simulink library "RS50_20S6P"  (R2025b)
settings: Solver=VariableStepAuto  StartTime=0.0  StopTime=10.0  RelTol=1e-3
undefined symbols (not defined in the file or in its folder): battery_builder_rtmsupport, gcbh
libraries: RS50_20S6P_lib x6
settings Model: Creator=oscar  LastModifiedBy=oscar

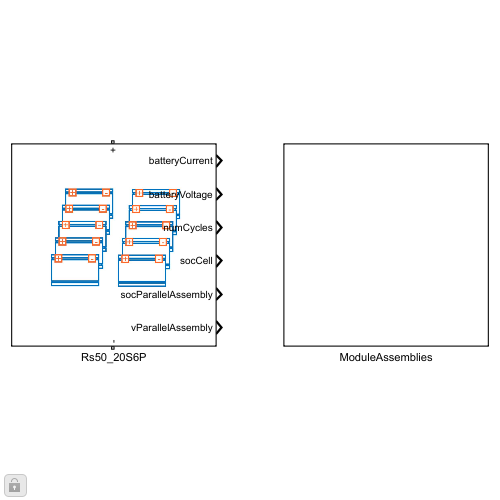
[thumbnail: Simulink's stored preview of the top-level diagram]
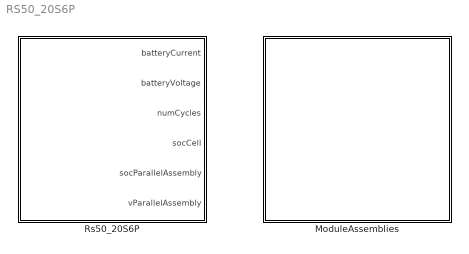
== system RS50_20S6P ==
  ModuleAssemblies : Subsystem
  Rs50_20S6P : Subsystem  LoadFcn=battery_builder_rtmsupport('loadfcn',gcbh);
      settings: CopyFcn=battery_builder_rtmsupport('copyfcn',gcbh);  PreCopyFcn=battery_builder_rtmsupport('precopyfcn',gcbh);  PreDeleteFcn=battery_builder_rtmsupport('predeletefcn',gcbh);  PortSchema="{\"entries\":[{\"content\":{\"sides\":[{\"content\":{\"connectorIds\":[\"LConn1\"]},\"type\":\"ConnectorPlacement.EquallySpacedRectSide\",\"uuid\":\"68108b1f-35ee-4bf1-8cf0-16152839d0de\"},{\"content\":{\"connectorIds\":[\"RConn1\"],\"side\":\"RIGHT\"},\"type\":\"ConnectorPlacement.EquallySpacedRectSide\",\"uuid\":\"9025f6ce-e211-4c4c-af6a-c12758361a55\"},{\"content\":{\"side\":\"TOP\"},\"type\":\"ConnectorPlacement.EquallySpacedRectSide\",\"uuid\":\"21b2816d-4a17-450d-8c21-7c5f468b8140\"},{\"content\":{\"connectorIds\":[\"Out1\",\"Out2\",\"Out3\",\"Out4\",\"Out5\",\"Out6\"],\"side\":\"BOTTOM\"},\"type\":\"ConnectorPlacement.EquallySpacedRectSide\",\"uuid\":\"2d886023-0113-46b2-8405-f6ad4fc498bb\"}]},\"type\":\"ConnectorPlacement.EquallySpacedConnector\",\"uuid\":\"b4619561-6c89-449f-a42b-64cd7bd240c0\"}],\"packageUris\":[\"http://schema.mathworks.com/mf0/Connector/R2020b\"],\"version\":\"1.0\"}"
      mask Display: image('$imagefile')

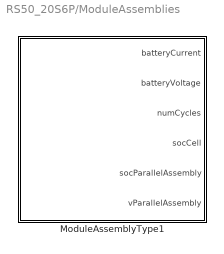
== system RS50_20S6P/ModuleAssemblies ==
  ModuleAssemblyType1 : Subsystem  LoadFcn=battery_builder_rtmsupport('loadfcn',gcbh);
      settings: CopyFcn=battery_builder_rtmsupport('copyfcn',gcbh);  PreCopyFcn=battery_builder_rtmsupport('precopyfcn',gcbh);  PreDeleteFcn=battery_builder_rtmsupport('predeletefcn',gcbh);  PortSchema="{\"entries\":[{\"content\":{\"sides\":[{\"content\":{\"connectorIds\":[\"LConn1\"]},\"type\":\"ConnectorPlacement.EquallySpacedRectSide\",\"uuid\":\"68108b1f-35ee-4bf1-8cf0-16152839d0de\"},{\"content\":{\"connectorIds\":[\"RConn1\"],\"side\":\"RIGHT\"},\"type\":\"ConnectorPlacement.EquallySpacedRectSide\",\"uuid\":\"9025f6ce-e211-4c4c-af6a-c12758361a55\"},{\"content\":{\"side\":\"TOP\"},\"type\":\"ConnectorPlacement.EquallySpacedRectSide\",\"uuid\":\"21b2816d-4a17-450d-8c21-7c5f468b8140\"},{\"content\":{\"connectorIds\":[\"Out1\",\"Out2\",\"Out3\",\"Out4\",\"Out5\",\"Out6\"],\"side\":\"BOTTOM\"},\"type\":\"ConnectorPlacement.EquallySpacedRectSide\",\"uuid\":\"a11e89a2-602c-4dcc-bda4-f5b907a63c99\"}]},\"type\":\"ConnectorPlacement.EquallySpacedConnector\",\"uuid\":\"b4619561-6c89-449f-a42b-64cd7bd240c0\"}],\"packageUris\":[\"http://schema.mathworks.com/mf0/Connector/R2020b\"],\"version\":\"1.0\"}"
      mask Display: image('$imagefile')

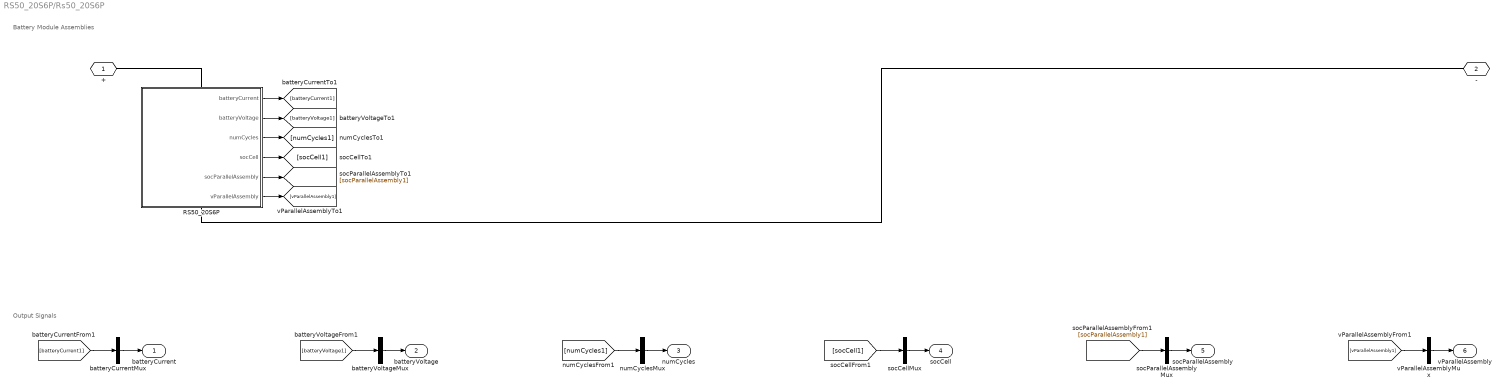
== system RS50_20S6P/Rs50_20S6P ==
  note: Battery Module Assemblies
  note: Output Signals
  RS50_20S6P : Subsystem  LoadFcn=battery_builder_rtmsupport('loadfcn',gcbh);
      settings: CopyFcn=battery_builder_rtmsupport('copyfcn',gcbh);  PreCopyFcn=battery_builder_rtmsupport('precopyfcn',gcbh);  PreDeleteFcn=battery_builder_rtmsupport('predeletefcn',gcbh);  PortSchema="{\"entries\":[{\"content\":{\"sides\":[{\"content\":{\"connectorIds\":[\"LConn1\"]},\"type\":\"ConnectorPlacement.EquallySpacedRectSide\",\"uuid\":\"68108b1f-35ee-4bf1-8cf0-16152839d0de\"},{\"content\":{\"connectorIds\":[\"RConn1\"],\"side\":\"RIGHT\"},\"type\":\"ConnectorPlacement.EquallySpacedRectSide\",\"uuid\":\"9025f6ce-e211-4c4c-af6a-c12758361a55\"},{\"content\":{\"side\":\"TOP\"},\"type\":\"ConnectorPlacement.EquallySpacedRectSide\",\"uuid\":\"21b2816d-4a17-450d-8c21-7c5f468b8140\"},{\"content\":{\"connectorIds\":[\"Out1\",\"Out2\",\"Out3\",\"Out4\",\"Out5\",\"Out6\"],\"side\":\"BOTTOM\"},\"type\":\"ConnectorPlacement.EquallySpacedRectSide\",\"uuid\":\"a11e89a2-602c-4dcc-bda4-f5b907a63c99\"}]},\"type\":\"ConnectorPlacement.EquallySpacedConnector\",\"uuid\":\"b4619561-6c89-449f-a42b-64cd7bd240c0\"}],\"packageUris\":[\"http://schema.mathworks.com/mf0/Connector/R2020b\"],\"version\":\"1.0\"}"
      mask Display: image('$imagefile')
  batteryCurrentMux : Mux  Inputs=1
  batteryVoltageMux : Mux  Inputs=1
  numCyclesMux : Mux  Inputs=1
  socCellMux : Mux  Inputs=1
  socParallelAssemblyMux : Mux  Inputs=1
  vParallelAssemblyMux : Mux  Inputs=1
  + : PMIOPort  Side=Left
  - : PMIOPort  Port=2  Side=Right
  batteryCurrent : Outport
  batteryVoltage : Outport  Port=2
  numCycles : Outport  Port=3
  socCell : Outport  Port=4
  socParallelAssembly : Outport  Port=5
  vParallelAssembly : Outport  Port=6
  wires:
  RS50_20S6P/1(batteryCurrent) -> [batteryCurrent1]
  batteryCurrentMux/1 -> batteryCurrent/1
  [batteryCurrent1] -> batteryCurrentMux/1
  RS50_20S6P/2(batteryVoltage) -> [batteryVoltage1]
  batteryVoltageMux/1 -> batteryVoltage/1
  [batteryVoltage1] -> batteryVoltageMux/1
  RS50_20S6P/3(numCycles) -> [numCycles1]
  numCyclesMux/1 -> numCycles/1
  [numCycles1] -> numCyclesMux/1
  RS50_20S6P/4(socCell) -> [socCell1]
  socCellMux/1 -> socCell/1
  [socCell1] -> socCellMux/1
  RS50_20S6P/5(socParallelAssembly) -> [socParallelAssembly1]
  socParallelAssemblyMux/1 -> socParallelAssembly/1
  [socParallelAssembly1] -> socParallelAssemblyMux/1
  RS50_20S6P/6(vParallelAssembly) -> [vParallelAssembly1]
  vParallelAssemblyMux/1 -> vParallelAssembly/1
  [vParallelAssembly1] -> vParallelAssemblyMux/1
  connections:
  RS50_20S6P/LConn1 -- +/RConn1
  RS50_20S6P/RConn1 -- -/RConn1

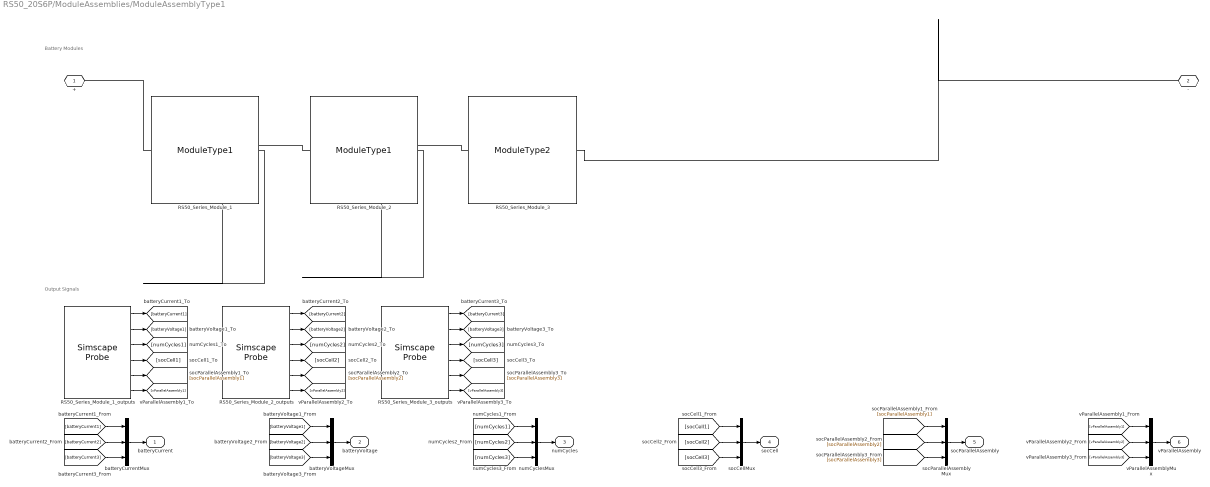
== system RS50_20S6P/ModuleAssemblies/ModuleAssemblyType1 ==
  note: Battery Modules
  note: Output Signals
  RS50_Series_Module_1 : RS50_20S6P_lib/Modules/ModuleType1  BatteryCapacityCell=27 A*hr  ExtrapolationMethodCell=simscape.enum.extrapolation.nearest  SOCBreakpointsCell=[0, .1, .25, .5, .75, .9, 1]  OpenCircuitVoltageCell=[3.5057, 3.566, 3.6337, 3.7127, 3.9259, 4.0777, 4.1928] V  VoltageRangeCell=[0, inf] V  ResistanceSOCBreakpointsCell=[0, .1, .25, .5, .75, .9, 1]  R0Cell=[.0085, .0085, .0087, .0082, .0083, .0085, .0085] Ohm  P=6  S=7  socCell_specify=off  socCell_priority=High  socCell=1  socCell_nominal_specify=off  socCell_nominal_value=1  socCell_nominal_unit=1  batteryVoltage_specify=off  batteryVoltage_priority=None  batteryVoltage=0 V  batteryVoltage_nominal_specify=off  batteryVoltage_nominal_value=1  batteryVoltage_nominal_unit=V  batteryCurrent_specify=off  batteryCurrent_priority=None  batteryCurrent=0 A  batteryCurrent_nominal_specify=off  batteryCurrent_nominal_value=1  batteryCurrent_nominal_unit=A  numCycles_specify=off  numCycles_priority=High  numCycles=0  numCycles_nominal_specify=off  numCycles_nominal_value=1  numCycles_nominal_unit=1  vParallelAssembly_specify=off  vParallelAssembly_priority=None  vParallelAssembly=repmat(0, 7, 1) V  vParallelAssembly_nominal_specify=off  vParallelAssembly_nominal_value=1  vParallelAssembly_nominal_unit=V  socParallelAssembly_specify=off  socParallelAssembly_priority=None  socParallelAssembly=repmat(1, 7, 1)  socParallelAssembly_nominal_specify=off  socParallelAssembly_nominal_value=1  socParallelAssembly_nominal_unit=1
      settings: InternalSimscapePortConfiguration="{\"Bottom\":[{\"id\":\"n\",\"label\":\"-\",\"type\":\"foundation.electrical.electrical\"}],\"Left\":[],\"Right\":[],\"Top\":[{\"id\":\"p\",\"label\":\"+\",\"type\":\"foundation.electrical.electrical\"}]}"
  RS50_Series_Module_1_outputs : SimscapeProbe  BoundBlock=3  Variables="{\"batteryCurrent\":{\"Probing\":\"ON\"},\"batteryVoltage\":{\"Probing\":\"ON\"},\"numCycles\":{\"Probing\":\"ON\"},\"socCell\":{\"Probing\":\"ON\"},\"socParallelAssembly\":{\"Probing\":\"ON\"},\"vParallelAssembly\":{\"Probing\":\"ON\"}}"
  RS50_Series_Module_2 : RS50_20S6P_lib/Modules/ModuleType1  BatteryCapacityCell=27 A*hr  ExtrapolationMethodCell=simscape.enum.extrapolation.nearest  SOCBreakpointsCell=[0, .1, .25, .5, .75, .9, 1]  OpenCircuitVoltageCell=[3.5057, 3.566, 3.6337, 3.7127, 3.9259, 4.0777, 4.1928] V  VoltageRangeCell=[0, inf] V  ResistanceSOCBreakpointsCell=[0, .1, .25, .5, .75, .9, 1]  R0Cell=[.0085, .0085, .0087, .0082, .0083, .0085, .0085] Ohm  P=6  S=7  socCell_specify=off  socCell_priority=High  socCell=1  socCell_nominal_specify=off  socCell_nominal_value=1  socCell_nominal_unit=1  batteryVoltage_specify=off  batteryVoltage_priority=None  batteryVoltage=0 V  batteryVoltage_nominal_specify=off  batteryVoltage_nominal_value=1  batteryVoltage_nominal_unit=V  batteryCurrent_specify=off  batteryCurrent_priority=None  batteryCurrent=0 A  batteryCurrent_nominal_specify=off  batteryCurrent_nominal_value=1  batteryCurrent_nominal_unit=A  numCycles_specify=off  numCycles_priority=High  numCycles=0  numCycles_nominal_specify=off  numCycles_nominal_value=1  numCycles_nominal_unit=1  vParallelAssembly_specify=off  vParallelAssembly_priority=None  vParallelAssembly=repmat(0, 7, 1) V  vParallelAssembly_nominal_specify=off  vParallelAssembly_nominal_value=1  vParallelAssembly_nominal_unit=V  socParallelAssembly_specify=off  socParallelAssembly_priority=None  socParallelAssembly=repmat(1, 7, 1)  socParallelAssembly_nominal_specify=off  socParallelAssembly_nominal_value=1  socParallelAssembly_nominal_unit=1
      settings: InternalSimscapePortConfiguration="{\"Bottom\":[{\"id\":\"n\",\"label\":\"-\",\"type\":\"foundation.electrical.electrical\"}],\"Left\":[],\"Right\":[],\"Top\":[{\"id\":\"p\",\"label\":\"+\",\"type\":\"foundation.electrical.electrical\"}]}"
  RS50_Series_Module_2_outputs : SimscapeProbe  BoundBlock=4  Variables="{\"batteryCurrent\":{\"Probing\":\"ON\"},\"batteryVoltage\":{\"Probing\":\"ON\"},\"numCycles\":{\"Probing\":\"ON\"},\"socCell\":{\"Probing\":\"ON\"},\"socParallelAssembly\":{\"Probing\":\"ON\"},\"vParallelAssembly\":{\"Probing\":\"ON\"}}"
  RS50_Series_Module_3 : RS50_20S6P_lib/Modules/ModuleType2  BatteryCapacityCell=27 A*hr  ExtrapolationMethodCell=simscape.enum.extrapolation.nearest  SOCBreakpointsCell=[0, .1, .25, .5, .75, .9, 1]  OpenCircuitVoltageCell=[3.5057, 3.566, 3.6337, 3.7127, 3.9259, 4.0777, 4.1928] V  VoltageRangeCell=[0, inf] V  ResistanceSOCBreakpointsCell=[0, .1, .25, .5, .75, .9, 1]  R0Cell=[.0085, .0085, .0087, .0082, .0083, .0085, .0085] Ohm  P=6  S=5  socCell_specify=off  socCell_priority=High  socCell=1  socCell_nominal_specify=off  socCell_nominal_value=1  socCell_nominal_unit=1  batteryVoltage_specify=off  batteryVoltage_priority=None  batteryVoltage=0 V  batteryVoltage_nominal_specify=off  batteryVoltage_nominal_value=1  batteryVoltage_nominal_unit=V  batteryCurrent_specify=off  batteryCurrent_priority=None  batteryCurrent=0 A  batteryCurrent_nominal_specify=off  batteryCurrent_nominal_value=1  batteryCurrent_nominal_unit=A  numCycles_specify=off  numCycles_priority=High  numCycles=0  numCycles_nominal_specify=off  numCycles_nominal_value=1  numCycles_nominal_unit=1  vParallelAssembly_specify=off  vParallelAssembly_priority=None  vParallelAssembly=repmat(0, 5, 1) V  vParallelAssembly_nominal_specify=off  vParallelAssembly_nominal_value=1  vParallelAssembly_nominal_unit=V  socParallelAssembly_specify=off  socParallelAssembly_priority=None  socParallelAssembly=repmat(1, 5, 1)  socParallelAssembly_nominal_specify=off  socParallelAssembly_nominal_value=1  socParallelAssembly_nominal_unit=1
      settings: InternalSimscapePortConfiguration="{\"Bottom\":[{\"id\":\"n\",\"label\":\"-\",\"type\":\"foundation.electrical.electrical\"}],\"Left\":[],\"Right\":[],\"Top\":[{\"id\":\"p\",\"label\":\"+\",\"type\":\"foundation.electrical.electrical\"}]}"
  RS50_Series_Module_3_outputs : SimscapeProbe  BoundBlock=5  Variables="{\"batteryCurrent\":{\"Probing\":\"ON\"},\"batteryVoltage\":{\"Probing\":\"ON\"},\"numCycles\":{\"Probing\":\"ON\"},\"socCell\":{\"Probing\":\"ON\"},\"socParallelAssembly\":{\"Probing\":\"ON\"},\"vParallelAssembly\":{\"Probing\":\"ON\"}}"
  batteryCurrentMux : Mux  Inputs=3
  batteryVoltageMux : Mux  Inputs=3
  numCyclesMux : Mux  Inputs=3
  socCellMux : Mux  Inputs=3
  socParallelAssemblyMux : Mux  Inputs=3
  vParallelAssemblyMux : Mux  Inputs=3
  + : PMIOPort  Side=Left
  - : PMIOPort  Port=2  Side=Right
  batteryCurrent : Outport
  batteryVoltage : Outport  Port=2
  numCycles : Outport  Port=3
  socCell : Outport  Port=4
  socParallelAssembly : Outport  Port=5
  vParallelAssembly : Outport  Port=6
  wires:
  RS50_Series_Module_1_outputs/1 -> [batteryCurrent1]
  batteryCurrentMux/1 -> batteryCurrent/1
  [batteryCurrent1] -> batteryCurrentMux/1
  RS50_Series_Module_1_outputs/2 -> [batteryVoltage1]
  batteryVoltageMux/1 -> batteryVoltage/1
  [batteryVoltage1] -> batteryVoltageMux/1
  RS50_Series_Module_1_outputs/3 -> [numCycles1]
  numCyclesMux/1 -> numCycles/1
  [numCycles1] -> numCyclesMux/1
  RS50_Series_Module_1_outputs/4 -> [socCell1]
  socCellMux/1 -> socCell/1
  [socCell1] -> socCellMux/1
  RS50_Series_Module_1_outputs/5 -> [socParallelAssembly1]
  socParallelAssemblyMux/1 -> socParallelAssembly/1
  [socParallelAssembly1] -> socParallelAssemblyMux/1
  RS50_Series_Module_1_outputs/6 -> [vParallelAssembly1]
  vParallelAssemblyMux/1 -> vParallelAssembly/1
  [vParallelAssembly1] -> vParallelAssemblyMux/1
  RS50_Series_Module_2_outputs/1 -> [batteryCurrent2]
  [batteryCurrent2] -> batteryCurrentMux/2
  RS50_Series_Module_2_outputs/2 -> [batteryVoltage2]
  [batteryVoltage2] -> batteryVoltageMux/2
  RS50_Series_Module_2_outputs/3 -> [numCycles2]
  [numCycles2] -> numCyclesMux/2
  RS50_Series_Module_2_outputs/4 -> [socCell2]
  [socCell2] -> socCellMux/2
  RS50_Series_Module_2_outputs/5 -> [socParallelAssembly2]
  [socParallelAssembly2] -> socParallelAssemblyMux/2
  RS50_Series_Module_2_outputs/6 -> [vParallelAssembly2]
  [vParallelAssembly2] -> vParallelAssemblyMux/2
  RS50_Series_Module_3_outputs/1 -> [batteryCurrent3]
  [batteryCurrent3] -> batteryCurrentMux/3
  RS50_Series_Module_3_outputs/2 -> [batteryVoltage3]
  [batteryVoltage3] -> batteryVoltageMux/3
  RS50_Series_Module_3_outputs/3 -> [numCycles3]
  [numCycles3] -> numCyclesMux/3
  RS50_Series_Module_3_outputs/4 -> [socCell3]
  [socCell3] -> socCellMux/3
  RS50_Series_Module_3_outputs/5 -> [socParallelAssembly3]
  [socParallelAssembly3] -> socParallelAssemblyMux/3
  RS50_Series_Module_3_outputs/6 -> [vParallelAssembly3]
  [vParallelAssembly3] -> vParallelAssemblyMux/3
  connections:
  RS50_Series_Module_2/LConn1 -- RS50_Series_Module_1/RConn1
  RS50_Series_Module_3/LConn1 -- RS50_Series_Module_2/RConn1
  RS50_Series_Module_1/LConn1 -- +/RConn1
  RS50_Series_Module_3/RConn1 -- -/RConn1

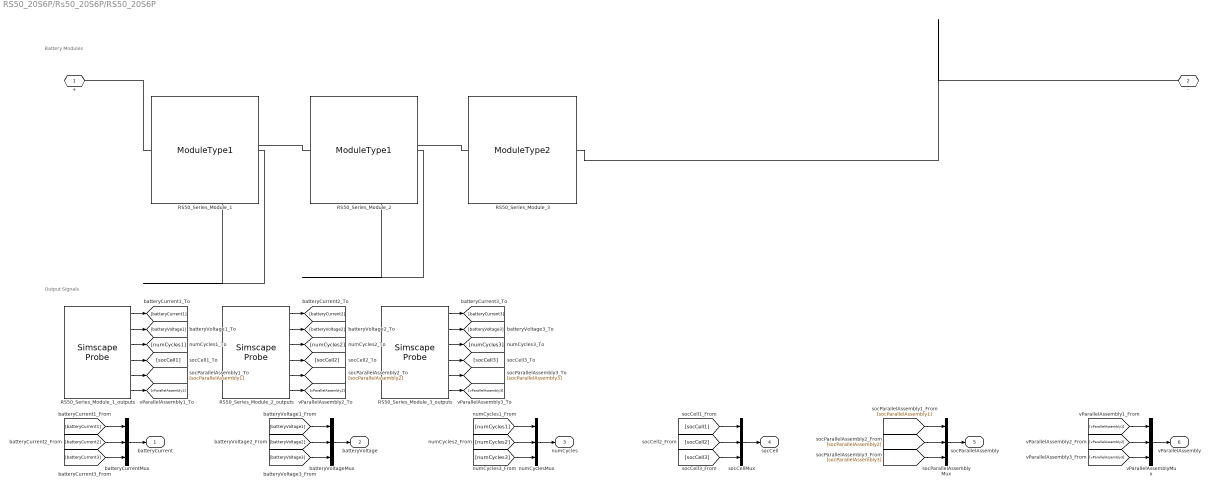
== system RS50_20S6P/Rs50_20S6P/RS50_20S6P ==
  note: Output Signals
  note: Battery Modules
  RS50_Series_Module_1 : RS50_20S6P_lib/Modules/ModuleType1  BatteryCapacityCell=27 A*hr  ExtrapolationMethodCell=simscape.enum.extrapolation.nearest  SOCBreakpointsCell=[0, .1, .25, .5, .75, .9, 1]  OpenCircuitVoltageCell=[3.5057, 3.566, 3.6337, 3.7127, 3.9259, 4.0777, 4.1928] V  VoltageRangeCell=[0, inf] V  ResistanceSOCBreakpointsCell=[0, .1, .25, .5, .75, .9, 1]  R0Cell=[.0085, .0085, .0087, .0082, .0083, .0085, .0085] Ohm  P=6  S=7  socCell_specify=off  socCell_priority=High  socCell=1  socCell_nominal_specify=off  socCell_nominal_value=1  socCell_nominal_unit=1  batteryVoltage_specify=off  batteryVoltage_priority=None  batteryVoltage=0 V  batteryVoltage_nominal_specify=off  batteryVoltage_nominal_value=1  batteryVoltage_nominal_unit=V  batteryCurrent_specify=off  batteryCurrent_priority=None  batteryCurrent=0 A  batteryCurrent_nominal_specify=off  batteryCurrent_nominal_value=1  batteryCurrent_nominal_unit=A  numCycles_specify=off  numCycles_priority=High  numCycles=0  numCycles_nominal_specify=off  numCycles_nominal_value=1  numCycles_nominal_unit=1  vParallelAssembly_specify=off  vParallelAssembly_priority=None  vParallelAssembly=repmat(0, 7, 1) V  vParallelAssembly_nominal_specify=off  vParallelAssembly_nominal_value=1  vParallelAssembly_nominal_unit=V  socParallelAssembly_specify=off  socParallelAssembly_priority=None  socParallelAssembly=repmat(1, 7, 1)  socParallelAssembly_nominal_specify=off  socParallelAssembly_nominal_value=1  socParallelAssembly_nominal_unit=1
      settings: InternalSimscapePortConfiguration="{\"Bottom\":[{\"id\":\"n\",\"label\":\"-\",\"type\":\"foundation.electrical.electrical\"}],\"Left\":[],\"Right\":[],\"Top\":[{\"id\":\"p\",\"label\":\"+\",\"type\":\"foundation.electrical.electrical\"}]}"
  RS50_Series_Module_1_outputs : SimscapeProbe  BoundBlock=63  Variables="{\"batteryCurrent\":{\"Probing\":\"ON\"},\"batteryVoltage\":{\"Probing\":\"ON\"},\"numCycles\":{\"Probing\":\"ON\"},\"socCell\":{\"Probing\":\"ON\"},\"socParallelAssembly\":{\"Probing\":\"ON\"},\"vParallelAssembly\":{\"Probing\":\"ON\"}}"
  RS50_Series_Module_2 : RS50_20S6P_lib/Modules/ModuleType1  BatteryCapacityCell=27 A*hr  ExtrapolationMethodCell=simscape.enum.extrapolation.nearest  SOCBreakpointsCell=[0, .1, .25, .5, .75, .9, 1]  OpenCircuitVoltageCell=[3.5057, 3.566, 3.6337, 3.7127, 3.9259, 4.0777, 4.1928] V  VoltageRangeCell=[0, inf] V  ResistanceSOCBreakpointsCell=[0, .1, .25, .5, .75, .9, 1]  R0Cell=[.0085, .0085, .0087, .0082, .0083, .0085, .0085] Ohm  P=6  S=7  socCell_specify=off  socCell_priority=High  socCell=1  socCell_nominal_specify=off  socCell_nominal_value=1  socCell_nominal_unit=1  batteryVoltage_specify=off  batteryVoltage_priority=None  batteryVoltage=0 V  batteryVoltage_nominal_specify=off  batteryVoltage_nominal_value=1  batteryVoltage_nominal_unit=V  batteryCurrent_specify=off  batteryCurrent_priority=None  batteryCurrent=0 A  batteryCurrent_nominal_specify=off  batteryCurrent_nominal_value=1  batteryCurrent_nominal_unit=A  numCycles_specify=off  numCycles_priority=High  numCycles=0  numCycles_nominal_specify=off  numCycles_nominal_value=1  numCycles_nominal_unit=1  vParallelAssembly_specify=off  vParallelAssembly_priority=None  vParallelAssembly=repmat(0, 7, 1) V  vParallelAssembly_nominal_specify=off  vParallelAssembly_nominal_value=1  vParallelAssembly_nominal_unit=V  socParallelAssembly_specify=off  socParallelAssembly_priority=None  socParallelAssembly=repmat(1, 7, 1)  socParallelAssembly_nominal_specify=off  socParallelAssembly_nominal_value=1  socParallelAssembly_nominal_unit=1
      settings: InternalSimscapePortConfiguration="{\"Bottom\":[{\"id\":\"n\",\"label\":\"-\",\"type\":\"foundation.electrical.electrical\"}],\"Left\":[],\"Right\":[],\"Top\":[{\"id\":\"p\",\"label\":\"+\",\"type\":\"foundation.electrical.electrical\"}]}"
  RS50_Series_Module_2_outputs : SimscapeProbe  BoundBlock=65  Variables="{\"batteryCurrent\":{\"Probing\":\"ON\"},\"batteryVoltage\":{\"Probing\":\"ON\"},\"numCycles\":{\"Probing\":\"ON\"},\"socCell\":{\"Probing\":\"ON\"},\"socParallelAssembly\":{\"Probing\":\"ON\"},\"vParallelAssembly\":{\"Probing\":\"ON\"}}"
  RS50_Series_Module_3 : RS50_20S6P_lib/Modules/ModuleType2  BatteryCapacityCell=27 A*hr  ExtrapolationMethodCell=simscape.enum.extrapolation.nearest  SOCBreakpointsCell=[0, .1, .25, .5, .75, .9, 1]  OpenCircuitVoltageCell=[3.5057, 3.566, 3.6337, 3.7127, 3.9259, 4.0777, 4.1928] V  VoltageRangeCell=[0, inf] V  ResistanceSOCBreakpointsCell=[0, .1, .25, .5, .75, .9, 1]  R0Cell=[.0085, .0085, .0087, .0082, .0083, .0085, .0085] Ohm  P=6  S=5  socCell_specify=off  socCell_priority=High  socCell=1  socCell_nominal_specify=off  socCell_nominal_value=1  socCell_nominal_unit=1  batteryVoltage_specify=off  batteryVoltage_priority=None  batteryVoltage=0 V  batteryVoltage_nominal_specify=off  batteryVoltage_nominal_value=1  batteryVoltage_nominal_unit=V  batteryCurrent_specify=off  batteryCurrent_priority=None  batteryCurrent=0 A  batteryCurrent_nominal_specify=off  batteryCurrent_nominal_value=1  batteryCurrent_nominal_unit=A  numCycles_specify=off  numCycles_priority=High  numCycles=0  numCycles_nominal_specify=off  numCycles_nominal_value=1  numCycles_nominal_unit=1  vParallelAssembly_specify=off  vParallelAssembly_priority=None  vParallelAssembly=repmat(0, 5, 1) V  vParallelAssembly_nominal_specify=off  vParallelAssembly_nominal_value=1  vParallelAssembly_nominal_unit=V  socParallelAssembly_specify=off  socParallelAssembly_priority=None  socParallelAssembly=repmat(1, 5, 1)  socParallelAssembly_nominal_specify=off  socParallelAssembly_nominal_value=1  socParallelAssembly_nominal_unit=1
      settings: InternalSimscapePortConfiguration="{\"Bottom\":[{\"id\":\"n\",\"label\":\"-\",\"type\":\"foundation.electrical.electrical\"}],\"Left\":[],\"Right\":[],\"Top\":[{\"id\":\"p\",\"label\":\"+\",\"type\":\"foundation.electrical.electrical\"}]}"
  RS50_Series_Module_3_outputs : SimscapeProbe  BoundBlock=67  Variables="{\"batteryCurrent\":{\"Probing\":\"ON\"},\"batteryVoltage\":{\"Probing\":\"ON\"},\"numCycles\":{\"Probing\":\"ON\"},\"socCell\":{\"Probing\":\"ON\"},\"socParallelAssembly\":{\"Probing\":\"ON\"},\"vParallelAssembly\":{\"Probing\":\"ON\"}}"
  batteryCurrentMux : Mux  Inputs=3
  batteryVoltageMux : Mux  Inputs=3
  numCyclesMux : Mux  Inputs=3
  socCellMux : Mux  Inputs=3
  socParallelAssemblyMux : Mux  Inputs=3
  vParallelAssemblyMux : Mux  Inputs=3
  + : PMIOPort  Side=Left
  - : PMIOPort  Port=2  Side=Right
  batteryCurrent : Outport
  batteryVoltage : Outport  Port=2
  numCycles : Outport  Port=3
  socCell : Outport  Port=4
  socParallelAssembly : Outport  Port=5
  vParallelAssembly : Outport  Port=6
  wires:
  [vParallelAssembly3] -> vParallelAssemblyMux/3
  RS50_Series_Module_3_outputs/6 -> [vParallelAssembly3]
  [socParallelAssembly3] -> socParallelAssemblyMux/3
  RS50_Series_Module_3_outputs/5 -> [socParallelAssembly3]
  [socCell3] -> socCellMux/3
  RS50_Series_Module_3_outputs/4 -> [socCell3]
  [numCycles3] -> numCyclesMux/3
  RS50_Series_Module_3_outputs/3 -> [numCycles3]
  [batteryVoltage3] -> batteryVoltageMux/3
  RS50_Series_Module_3_outputs/2 -> [batteryVoltage3]
  [batteryCurrent3] -> batteryCurrentMux/3
  RS50_Series_Module_3_outputs/1 -> [batteryCurrent3]
  [vParallelAssembly2] -> vParallelAssemblyMux/2
  RS50_Series_Module_2_outputs/6 -> [vParallelAssembly2]
  [socParallelAssembly2] -> socParallelAssemblyMux/2
  RS50_Series_Module_2_outputs/5 -> [socParallelAssembly2]
  [socCell2] -> socCellMux/2
  RS50_Series_Module_2_outputs/4 -> [socCell2]
  [numCycles2] -> numCyclesMux/2
  RS50_Series_Module_2_outputs/3 -> [numCycles2]
  [batteryVoltage2] -> batteryVoltageMux/2
  RS50_Series_Module_2_outputs/2 -> [batteryVoltage2]
  [batteryCurrent2] -> batteryCurrentMux/2
  RS50_Series_Module_2_outputs/1 -> [batteryCurrent2]
  [vParallelAssembly1] -> vParallelAssemblyMux/1
  vParallelAssemblyMux/1 -> vParallelAssembly/1
  RS50_Series_Module_1_outputs/6 -> [vParallelAssembly1]
  [socParallelAssembly1] -> socParallelAssemblyMux/1
  socParallelAssemblyMux/1 -> socParallelAssembly/1
  RS50_Series_Module_1_outputs/5 -> [socParallelAssembly1]
  [socCell1] -> socCellMux/1
  socCellMux/1 -> socCell/1
  RS50_Series_Module_1_outputs/4 -> [socCell1]
  [numCycles1] -> numCyclesMux/1
  numCyclesMux/1 -> numCycles/1
  RS50_Series_Module_1_outputs/3 -> [numCycles1]
  [batteryVoltage1] -> batteryVoltageMux/1
  batteryVoltageMux/1 -> batteryVoltage/1
  RS50_Series_Module_1_outputs/2 -> [batteryVoltage1]
  [batteryCurrent1] -> batteryCurrentMux/1
  batteryCurrentMux/1 -> batteryCurrent/1
  RS50_Series_Module_1_outputs/1 -> [batteryCurrent1]
  connections:
  RS50_Series_Module_3/RConn1 -- -/RConn1
  RS50_Series_Module_1/LConn1 -- +/RConn1
  RS50_Series_Module_3/LConn1 -- RS50_Series_Module_2/RConn1
  RS50_Series_Module_2/LConn1 -- RS50_Series_Module_1/RConn1
